simulink model "full_three_axis"  (R2026b)
settings: Solver=VariableStepAuto  StopTime=2
undefined symbols (not defined in the file): Bambient, k, T_threshold, Vmax
libraries: stm32f4xxblockslib x20, simulink x3, slpidlib x3, stm32blockslib x2, stm32g4xxblockslib x2
settings Model: STM32="{\"PWMOutput\":[{\"ID\":\"308\"},{\"ID\":\"321\"},{\"ID\":\"322\"}],\"UARTRead\":{\"ID\":\"291\"},\"AnalogInput\":{\"ID\":\"326\"},\"DigitalPortRead\":[{\"ID\":\"328\"},{\"ID\":\"404\"},{\"ID\":\"509\"},{\"ID\":\"514\"},{\"ID\":\"520\"},{\"ID\":\"525\"}],\"DigitalPortWrite\":[{\"ID\":\"353\"},{\"ID\":\"325\"},{\"ID\":\"370\"},{\"ID\":\"495\"},{\"ID\":\"497\"},{\"ID\":\"519\"},{\"ID\":\"530\"},{\"ID\":\"532\"},{\"ID\":\"534\"}],\"HardwareInterrupt\":[{\"ID\":\"333\"},{\"ID\":\"334\"}],\"UARTWrite\":{\"ID\":\"545\"}}"  Creator=Samuel  LastModifiedBy=Samuel
settings SimscapeCC: SimscapeUseEnergyAccounting=off

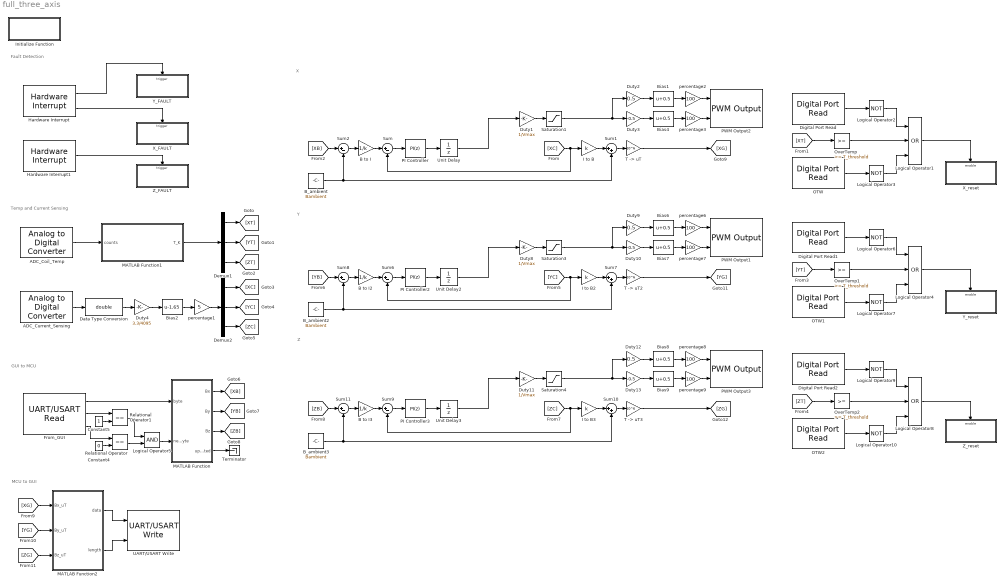
== system full_three_axis ==
  note: MCU to GUI
  note: Z
  note: Y
  note: X
  note: GUI to MCU
  note: Fault Detection
  note: Temp and Current Sensing
  ADC_Coil_Temp : stm32f4xxblockslib/Analog to Digital Converter  ADCModule=ADC2  ConversionGroup=Regular  TriggerMode=Trigger and read  NumberOfConversions=3  EnableBufferConv=off  BufferLength=1  OutputStatus=off  SampleTime=0.001  EnableSimPort=off  hoistedMaskSrc=ECSoC/ECSimCodegen/Analog to Digital Converter
  ADC_Current_Sensing : stm32f4xxblockslib/Analog to Digital Converter  ADCModule=ADC1  ConversionGroup=Regular  TriggerMode=Trigger and read  NumberOfConversions=3  EnableBufferConv=off  BufferLength=1  OutputStatus=off  SampleTime=0.001  EnableSimPort=off  hoistedMaskSrc=ECSoC/ECSimCodegen/Analog to Digital Converter
  B to I : Gain  Gain=1/k
  B to I2 : Gain  Gain=1/k
  B to I3 : Gain  Gain=1/k
  B_ambient : Constant  Value=Bambient
  B_ambient2 : Constant  Value=Bambient
  B_ambient3 : Constant  Value=Bambient
  Bias{1,4,6..9} (6 alike) : Bias  Bias=0.5  SaturateOnIntegerOverflow=off
  Bias2 : Bias  Bias=-1.65  SaturateOnIntegerOverflow=off
  Constant4 : Constant  Value=0
  Constant5 : Constant
  Data Type Conversion : DataTypeConversion  OutDataTypeStr=double  SaturateOnIntegerOverflow=off  RndMeth=Floor
  Demux1 : Demux  Outputs=3
  Demux2 : Demux  Outputs=3
  Digital Port Read : stm32f4xxblockslib/Digital Port Read  PortName=GPIOB  PinNumber=12  ReadOperation=on  IOAsArray=off  SampleTime=0.001  EnableSimPort=off  hoistedMaskSrc=ECSoC/ECSimCodegen/Digital Port Read
      settings: LibrarySourceBlock=stm32g4xxblockslib/Digital Port Read
  Digital Port Read1 : stm32f4xxblockslib/Digital Port Read  PortName=GPIOB  PinNumber=15  ReadOperation=on  IOAsArray=off  SampleTime=0.001  EnableSimPort=off  hoistedMaskSrc=ECSoC/ECSimCodegen/Digital Port Read
      settings: LibrarySourceBlock=stm32g4xxblockslib/Digital Port Read
  Digital Port Read2 : stm32f4xxblockslib/Digital Port Read  PortName=GPIOB  PinNumber=2  ReadOperation=on  IOAsArray=off  SampleTime=0.001  EnableSimPort=off  hoistedMaskSrc=ECSoC/ECSimCodegen/Digital Port Read
      settings: LibrarySourceBlock=stm32g4xxblockslib/Digital Port Read
  Duty1 : Gain  Gain=1/Vmax
  Duty10 : Gain  Gain=-0.5
  Duty11 : Gain  Gain=1/Vmax
  Duty12 : Gain  Gain=0.5
  Duty13 : Gain  Gain=-0.5
  Duty2 : Gain  Gain=0.5
  Duty3 : Gain  Gain=-0.5
  Duty4 : Gain  Gain=3.3/4095
  Duty8 : Gain  Gain=1/Vmax
  Duty9 : Gain  Gain=0.5
  From_GUI : stm32blockslib/UART//USART Read  UARTModule=LPUART1  DataType=uint8  DataLength=1  BlockingMode=off  BlockingTimeout=0.1  OutputLength=on  OutputStatus=on  SampleTime=0.001
  Hardware Interrupt : stm32g4xxblockslib/Hardware Interrupt  ISRGroup=External interrupts (EXTI)  ISRName=EXTI15_10_IRQHandler  ISRFunctionName=EXTI15_10_IRQHandler  ISRNumber=55  TaskPriority=30  EventsList={ 'on', 'EXTI15 Event', '1', 'inherit', 'off'; 'off', 'EXTI14 Event', '2', 'inherit', 'off'; 'off', 'EXTI13 Event', '3', 'inherit', 'off'; 'on', 'EXTI12 Event', '4', 'inherit', 'off'; 'off', 'EXTI11 Event', '5', 'inherit', 'off'; 'off', 'EXTI10 Event', '6', 'inherit', 'off'; 'off', 'Custom event', '7', 'inherit', 'off' }  SelectedEvents={'EXTI15 Event','EXTI12 Event'}  InternalTaskPriority=30  DisablePreemption=off  ClearInterruptFlagsAtEndOfEvent=on  InterruptDefinitionFile=$(TARGET_ROOT)/registry/interrupts/STM32F4xxBased_interrupts.xml  HardwareBoard=STM32G4xx Based  EnableSimPort=off
  Hardware Interrupt1 : stm32g4xxblockslib/Hardware Interrupt  ISRGroup=External interrupts (EXTI)  ISRName=EXTI2_IRQHandler  ISRFunctionName=EXTI2_IRQHandler  ISRNumber=23  TaskPriority=30  EventsList={ 'on', 'EXTI2 Event', '1', 'inherit', 'off'; 'off', 'Custom event', '2', 'inherit', 'off' }  SelectedEvents={'EXTI2 Event'}  InternalTaskPriority=30  DisablePreemption=off  ClearInterruptFlagsAtEndOfEvent=on  InterruptDefinitionFile=$(TARGET_ROOT)/registry/interrupts/STM32F4xxBased_interrupts.xml  HardwareBoard=STM32G4xx Based  EnableSimPort=off
  I to B : Gain  Gain=k
  I to B2 : Gain  Gain=k
  I to B3 : Gain  Gain=k
  Initialize Function : Subsystem  TreatAsAtomicUnit=on
  Logical Operator1 : Logic  Operator=OR  Inputs=3  AllPortsSameDT=off  OutDataTypeStr=boolean
  Logical Operator{2..3,6..7,9..10} (6 alike) : Logic  Operator=NOT  AllPortsSameDT=off  OutDataTypeStr=boolean
  Logical Operator4 : Logic  Operator=OR  Inputs=3  AllPortsSameDT=off  OutDataTypeStr=boolean
  Logical Operator5 : Logic  AllPortsSameDT=off  OutDataTypeStr=boolean
  Logical Operator8 : Logic  Operator=OR  Inputs=3  AllPortsSameDT=off  OutDataTypeStr=boolean
  MATLAB Function : MATLAB Function  TreatAsAtomicUnit=on
  MATLAB Function1 : MATLAB Function  TreatAsAtomicUnit=on
  MATLAB Function2 : MATLAB Function  TreatAsAtomicUnit=on
  OTW : stm32f4xxblockslib/Digital Port Read  PortName=GPIOB  PinNumber=11  ReadOperation=on  IOAsArray=off  SampleTime=0.001  EnableSimPort=off  hoistedMaskSrc=ECSoC/ECSimCodegen/Digital Port Read
      settings: LibrarySourceBlock=stm32g4xxblockslib/Digital Port Read
  OTW1 : stm32f4xxblockslib/Digital Port Read  PortName=GPIOB  PinNumber=14  ReadOperation=on  IOAsArray=off  SampleTime=0.001  EnableSimPort=off  hoistedMaskSrc=ECSoC/ECSimCodegen/Digital Port Read
      settings: LibrarySourceBlock=stm32g4xxblockslib/Digital Port Read
  OTW2 : stm32f4xxblockslib/Digital Port Read  PortName=GPIOB  PinNumber=1  ReadOperation=on  IOAsArray=off  SampleTime=0.001  EnableSimPort=off  hoistedMaskSrc=ECSoC/ECSimCodegen/Digital Port Read
      settings: LibrarySourceBlock=stm32g4xxblockslib/Digital Port Read
  OverTemp : simulink/Logic and Bit Operations/Compare To Constant  relop=>=  const=T_threshold  OutDataTypeStr=boolean
  OverTemp1 : simulink/Logic and Bit Operations/Compare To Constant  relop=>=  const=T_threshold  OutDataTypeStr=boolean
  OverTemp2 : simulink/Logic and Bit Operations/Compare To Constant  relop=>=  const=T_threshold  OutDataTypeStr=boolean
  PI Controller : slpidlib/PID Controller  Controller=PI  Form=Parallel  TimeDomain=Discrete-time  UseExternalTs=off  SampleTime=1e-4  IntegratorMethod=Forward Euler  FilterMethod=Forward Euler  ControllerParametersSource=internal  P=5  I=200  UseKiTs=off  D=0  UseExternalDerivativeSource=off  N=100  UseFilter=on  TunerSelectOption=Transfer Function Based (PID Tuner App)  InitialConditionSource=internal  InitialConditionForIntegrator=0  InitialConditionForFilter=0  DifferentiatorICPrevScaledInput=0  ExternalReset=none  TrackingMode=off  Kt=1  LimitOutput=on  SatLimitsSource=internal  UpperSaturationLimit=30  LowerSaturationLimit=-30  LinearizeAsGain=on  AntiWindupMode=clamping  Kb=1  LimitIntegrator=off  UpperIntegratorSaturationLimit=inf  LowerIntegratorSaturationLimit=-inf  POutMin=[]  POutMax=[]  IOutMin=[]  IOutMax=[]  DOutMin=[]  DOutMax=[]  NOutMin=[]  NOutMax=[]  SumOutMin=[]  SumOutMax=[]  SaturationOutMin=[]  SaturationOutMax=[]  PParamMin=[]  PParamMax=[]  IParamMin=[]  IParamMax=[]  DParamMin=[]  DParamMax=[]  NParamMin=[]  NParamMax=[]  KbParamMin=[]  KbParamMax=[]  KtParamMin=[]  KtParamMax=[]  KbOutMin=[]  KbOutMax=[]  KtOutMin=[]  KtOutMax=[]  IntegratorOutMin=[]  IntegratorOutMax=[]  FilterOutMin=[]  FilterOutMax=[]  SumI1OutMin=[]  SumI1OutMax=[]  SumI2OutMin=[]  SumI2OutMax=[]  SumI3OutMin=[]  SumI3OutMax=[]  SumI4OutMin=[]  SumI4OutMax=[]  SumDOutMin=[]  SumDOutMax=[]  DifferentiatorOutMin=[]  DifferentiatorOutMax=[]  FilterDiffOutCoefMin=[]  FilterDiffOutCoefMax=[]  ReciprocalOutMin=[]  ReciprocalOutMax=[]  SumDenOutMin=[]  SumDenOutMax=[]  SumNumOutMin=[]  SumNumOutMax=[]  DivideOutMin=[]  DivideOutMax=[]  UdiffTsProdOutMin=[]  UdiffTsProdOutMax=[]  NTsProdOutMin=[]  NTsProdOutMax=[]  UintegralTsProdOutMin=[]  UintegralTsProdOutMax=[]  UngainTsProdOutMin=[]  UngainTsProdOutMax=[]  ClampingZeroOutDataTypeStr=Inherit: Inherit via back propagation  ClampingZeroOutMin=[]  ClampingZeroOutMax=[]  FilterDenConstantOutDataTypeStr=Inherit: Inherit via back propagation  FilterDenConstantOutMin=[]  FilterDenConstantOutMax=[]  PCopyOutDataTypeStr=Inherit: Inherit via back propagation  PCopyOutMin=[]  PCopyOutMax=[]  NCopyOutDataTypeStr=Inherit: Inherit via back propagation  NCopyOutMin=[]  NCopyOutMax=[]  IntegratorContinuousStateAttributes=''  IntegratorStateMustResolveToSignalObject=off  IntegratorRTWStateStorageClass=Auto  FilterContinuousStateAttributes=''  FilterStateMustResolveToSignalObject=off  FilterRTWStateStorageClass=Auto  ParallelPVariant=InternalParameters  IdealPVariant=Disabled  IVariant=InternalParameters  DVariant=Disabled  IntegratorVariant=Discrete  SatVariant=Enabled  AWVariant=DiscClampingParallel  PCopyVariant=Disabled  TRVariant=Disabled  FdbkBlocksVariant=Forward  IdealPFdbkVariant=Disabled  SatFdbkVariant=Disabled  DerivativeFilterVariant=Disabled  NVariant=Disabled  NCopyVariant=Disabled_SignalSpec  FilterICVariant=Disabled  IntegratorICVariant=InternalICs  ExternalResetVariant=Disabled  TRSumVariant=Passthrough  SumFdbkVariant=Disabled  SumVariant=Sum_PI  TsampFilterVariant=InternalTs  TsampNgainVariant=Passthrough  TsampIntegralVariant=Disabled_SignalSpec  ExternalSaturationOutDataTypeStr=Inherit: Same as second input  DerivativeSourceVariant=Disabled  PreIntVariant=InternalPreInt
  PI Controller2 : slpidlib/PID Controller  Controller=PI  Form=Parallel  TimeDomain=Discrete-time  UseExternalTs=off  SampleTime=1e-4  IntegratorMethod=Forward Euler  FilterMethod=Forward Euler  ControllerParametersSource=internal  P=5  I=200  UseKiTs=off  D=0  UseExternalDerivativeSource=off  N=100  UseFilter=on  TunerSelectOption=Transfer Function Based (PID Tuner App)  InitialConditionSource=internal  InitialConditionForIntegrator=0  InitialConditionForFilter=0  DifferentiatorICPrevScaledInput=0  ExternalReset=none  TrackingMode=off  Kt=1  LimitOutput=on  SatLimitsSource=internal  UpperSaturationLimit=30  LowerSaturationLimit=-30  LinearizeAsGain=on  AntiWindupMode=clamping  Kb=1  LimitIntegrator=off  UpperIntegratorSaturationLimit=inf  LowerIntegratorSaturationLimit=-inf  POutMin=[]  POutMax=[]  IOutMin=[]  IOutMax=[]  DOutMin=[]  DOutMax=[]  NOutMin=[]  NOutMax=[]  SumOutMin=[]  SumOutMax=[]  SaturationOutMin=[]  SaturationOutMax=[]  PParamMin=[]  PParamMax=[]  IParamMin=[]  IParamMax=[]  DParamMin=[]  DParamMax=[]  NParamMin=[]  NParamMax=[]  KbParamMin=[]  KbParamMax=[]  KtParamMin=[]  KtParamMax=[]  KbOutMin=[]  KbOutMax=[]  KtOutMin=[]  KtOutMax=[]  IntegratorOutMin=[]  IntegratorOutMax=[]  FilterOutMin=[]  FilterOutMax=[]  SumI1OutMin=[]  SumI1OutMax=[]  SumI2OutMin=[]  SumI2OutMax=[]  SumI3OutMin=[]  SumI3OutMax=[]  SumI4OutMin=[]  SumI4OutMax=[]  SumDOutMin=[]  SumDOutMax=[]  DifferentiatorOutMin=[]  DifferentiatorOutMax=[]  FilterDiffOutCoefMin=[]  FilterDiffOutCoefMax=[]  ReciprocalOutMin=[]  ReciprocalOutMax=[]  SumDenOutMin=[]  SumDenOutMax=[]  SumNumOutMin=[]  SumNumOutMax=[]  DivideOutMin=[]  DivideOutMax=[]  UdiffTsProdOutMin=[]  UdiffTsProdOutMax=[]  NTsProdOutMin=[]  NTsProdOutMax=[]  UintegralTsProdOutMin=[]  UintegralTsProdOutMax=[]  UngainTsProdOutMin=[]  UngainTsProdOutMax=[]  ClampingZeroOutDataTypeStr=Inherit: Inherit via back propagation  ClampingZeroOutMin=[]  ClampingZeroOutMax=[]  FilterDenConstantOutDataTypeStr=Inherit: Inherit via back propagation  FilterDenConstantOutMin=[]  FilterDenConstantOutMax=[]  PCopyOutDataTypeStr=Inherit: Inherit via back propagation  PCopyOutMin=[]  PCopyOutMax=[]  NCopyOutDataTypeStr=Inherit: Inherit via back propagation  NCopyOutMin=[]  NCopyOutMax=[]  IntegratorContinuousStateAttributes=''  IntegratorStateMustResolveToSignalObject=off  IntegratorRTWStateStorageClass=Auto  FilterContinuousStateAttributes=''  FilterStateMustResolveToSignalObject=off  FilterRTWStateStorageClass=Auto  ParallelPVariant=InternalParameters  IdealPVariant=Disabled  IVariant=InternalParameters  DVariant=Disabled  IntegratorVariant=Discrete  SatVariant=Enabled  AWVariant=DiscClampingParallel  PCopyVariant=Disabled  TRVariant=Disabled  FdbkBlocksVariant=Forward  IdealPFdbkVariant=Disabled  SatFdbkVariant=Disabled  DerivativeFilterVariant=Disabled  NVariant=Disabled  NCopyVariant=Disabled_SignalSpec  FilterICVariant=Disabled  IntegratorICVariant=InternalICs  ExternalResetVariant=Disabled  TRSumVariant=Passthrough  SumFdbkVariant=Disabled  SumVariant=Sum_PI  TsampFilterVariant=InternalTs  TsampNgainVariant=Passthrough  TsampIntegralVariant=Disabled_SignalSpec  ExternalSaturationOutDataTypeStr=Inherit: Same as second input  DerivativeSourceVariant=Disabled  PreIntVariant=InternalPreInt
  PI Controller3 : slpidlib/PID Controller  Controller=PI  Form=Parallel  TimeDomain=Discrete-time  UseExternalTs=off  SampleTime=1e-4  IntegratorMethod=Forward Euler  FilterMethod=Forward Euler  ControllerParametersSource=internal  P=5  I=200  UseKiTs=off  D=0  UseExternalDerivativeSource=off  N=100  UseFilter=on  TunerSelectOption=Transfer Function Based (PID Tuner App)  InitialConditionSource=internal  InitialConditionForIntegrator=0  InitialConditionForFilter=0  DifferentiatorICPrevScaledInput=0  ExternalReset=none  TrackingMode=off  Kt=1  LimitOutput=on  SatLimitsSource=internal  UpperSaturationLimit=30  LowerSaturationLimit=-30  LinearizeAsGain=on  AntiWindupMode=clamping  Kb=1  LimitIntegrator=off  UpperIntegratorSaturationLimit=inf  LowerIntegratorSaturationLimit=-inf  POutMin=[]  POutMax=[]  IOutMin=[]  IOutMax=[]  DOutMin=[]  DOutMax=[]  NOutMin=[]  NOutMax=[]  SumOutMin=[]  SumOutMax=[]  SaturationOutMin=[]  SaturationOutMax=[]  PParamMin=[]  PParamMax=[]  IParamMin=[]  IParamMax=[]  DParamMin=[]  DParamMax=[]  NParamMin=[]  NParamMax=[]  KbParamMin=[]  KbParamMax=[]  KtParamMin=[]  KtParamMax=[]  KbOutMin=[]  KbOutMax=[]  KtOutMin=[]  KtOutMax=[]  IntegratorOutMin=[]  IntegratorOutMax=[]  FilterOutMin=[]  FilterOutMax=[]  SumI1OutMin=[]  SumI1OutMax=[]  SumI2OutMin=[]  SumI2OutMax=[]  SumI3OutMin=[]  SumI3OutMax=[]  SumI4OutMin=[]  SumI4OutMax=[]  SumDOutMin=[]  SumDOutMax=[]  DifferentiatorOutMin=[]  DifferentiatorOutMax=[]  FilterDiffOutCoefMin=[]  FilterDiffOutCoefMax=[]  ReciprocalOutMin=[]  ReciprocalOutMax=[]  SumDenOutMin=[]  SumDenOutMax=[]  SumNumOutMin=[]  SumNumOutMax=[]  DivideOutMin=[]  DivideOutMax=[]  UdiffTsProdOutMin=[]  UdiffTsProdOutMax=[]  NTsProdOutMin=[]  NTsProdOutMax=[]  UintegralTsProdOutMin=[]  UintegralTsProdOutMax=[]  UngainTsProdOutMin=[]  UngainTsProdOutMax=[]  ClampingZeroOutDataTypeStr=Inherit: Inherit via back propagation  ClampingZeroOutMin=[]  ClampingZeroOutMax=[]  FilterDenConstantOutDataTypeStr=Inherit: Inherit via back propagation  FilterDenConstantOutMin=[]  FilterDenConstantOutMax=[]  PCopyOutDataTypeStr=Inherit: Inherit via back propagation  PCopyOutMin=[]  PCopyOutMax=[]  NCopyOutDataTypeStr=Inherit: Inherit via back propagation  NCopyOutMin=[]  NCopyOutMax=[]  IntegratorContinuousStateAttributes=''  IntegratorStateMustResolveToSignalObject=off  IntegratorRTWStateStorageClass=Auto  FilterContinuousStateAttributes=''  FilterStateMustResolveToSignalObject=off  FilterRTWStateStorageClass=Auto  ParallelPVariant=InternalParameters  IdealPVariant=Disabled  IVariant=InternalParameters  DVariant=Disabled  IntegratorVariant=Discrete  SatVariant=Enabled  AWVariant=DiscClampingParallel  PCopyVariant=Disabled  TRVariant=Disabled  FdbkBlocksVariant=Forward  IdealPFdbkVariant=Disabled  SatFdbkVariant=Disabled  DerivativeFilterVariant=Disabled  NVariant=Disabled  NCopyVariant=Disabled_SignalSpec  FilterICVariant=Disabled  IntegratorICVariant=InternalICs  ExternalResetVariant=Disabled  TRSumVariant=Passthrough  SumFdbkVariant=Disabled  SumVariant=Sum_PI  TsampFilterVariant=InternalTs  TsampNgainVariant=Passthrough  TsampIntegralVariant=Disabled_SignalSpec  ExternalSaturationOutDataTypeStr=Inherit: Same as second input  DerivativeSourceVariant=Disabled  PreIntVariant=InternalPreInt
  PWM Output1 : stm32f4xxblockslib/PWM Output  ProcessorFamily=STM32G4  TimerModule=TIM1  DutycycleUnits=Percentage  EnableChannel1=off  EnableCaptureCompare1Input=off  EnableCaptureCompare1ComplementaryInput=off  EnableOutputCompare1ModeInput=off  EnableChannel2=off  EnableCaptureCompare2Input=off  EnableCaptureCompare2ComplementaryInput=off  EnableOutputCompare2ModeInput=off  EnableChannel3=on  EnableCaptureCompare3Input=off  EnableCaptureCompare3ComplementaryInput=off  EnableOutputCompare3ModeInput=off  EnableChannel4=on  EnableCaptureCompare4Input=off  EnableCaptureCompare4ComplementaryInput=off  EnableOutputCompare4ModeInput=off  EnableChannel5=off  EnableCaptureCompare5Input=off  EnableOutputCompare5ModeInput=off  EnableChannel6=off  EnableCaptureCompare6Input=off  EnableOutputCompare6ModeInput=off  EnableCounterInput=off  EnableMainOutputInput=off  EnableFrequencyInput=off  SetRCAfterCE=off  OutputDirection=off  OutputMainOutputEnableStatus=off  SampleTime=0.1  EnableSimPort=off  EnableUpdateEvent=off  EnableCaptureCompare1Event=off  EnableCaptureCompare2Event=off  EnableCaptureCompare3Event=off  EnableCaptureCompare4Event=off  EnableTriggerEvent=off  EnableBreakEvent=off  EnableBreakEvent2=off  hoistedMaskSrc=ECSoC/ECSimCodegen/PWM Output
      settings: LibrarySourceBlock=stm32g4xxblockslib/PWM Output
  PWM Output2 : stm32f4xxblockslib/PWM Output  ProcessorFamily=STM32G4  TimerModule=TIM1  DutycycleUnits=Percentage  EnableChannel1=on  EnableCaptureCompare1Input=off  EnableCaptureCompare1ComplementaryInput=off  EnableOutputCompare1ModeInput=off  EnableChannel2=on  EnableCaptureCompare2Input=off  EnableCaptureCompare2ComplementaryInput=off  EnableOutputCompare2ModeInput=off  EnableChannel3=off  EnableCaptureCompare3Input=off  EnableCaptureCompare3ComplementaryInput=off  EnableOutputCompare3ModeInput=off  EnableChannel4=off  EnableCaptureCompare4Input=off  EnableCaptureCompare4ComplementaryInput=off  EnableOutputCompare4ModeInput=off  EnableChannel5=off  EnableCaptureCompare5Input=off  EnableOutputCompare5ModeInput=off  EnableChannel6=off  EnableCaptureCompare6Input=off  EnableOutputCompare6ModeInput=off  EnableCounterInput=off  EnableMainOutputInput=off  EnableFrequencyInput=off  SetRCAfterCE=off  OutputDirection=off  OutputMainOutputEnableStatus=off  SampleTime=0.1  EnableSimPort=off  EnableUpdateEvent=off  EnableCaptureCompare1Event=off  EnableCaptureCompare2Event=off  EnableCaptureCompare3Event=off  EnableCaptureCompare4Event=off  EnableTriggerEvent=off  EnableBreakEvent=off  EnableBreakEvent2=off  hoistedMaskSrc=ECSoC/ECSimCodegen/PWM Output
      settings: LibrarySourceBlock=stm32g4xxblockslib/PWM Output
  PWM Output3 : stm32f4xxblockslib/PWM Output  ProcessorFamily=STM32G4  TimerModule=TIM8  DutycycleUnits=Percentage  EnableChannel1=on  EnableCaptureCompare1Input=off  EnableCaptureCompare1ComplementaryInput=off  EnableOutputCompare1ModeInput=off  EnableChannel2=on  EnableCaptureCompare2Input=off  EnableCaptureCompare2ComplementaryInput=off  EnableOutputCompare2ModeInput=off  EnableChannel3=off  EnableCaptureCompare3Input=off  EnableCaptureCompare3ComplementaryInput=off  EnableOutputCompare3ModeInput=off  EnableChannel4=off  EnableCaptureCompare4Input=off  EnableCaptureCompare4ComplementaryInput=off  EnableOutputCompare4ModeInput=off  EnableChannel5=off  EnableCaptureCompare5Input=off  EnableOutputCompare5ModeInput=off  EnableChannel6=off  EnableCaptureCompare6Input=off  EnableOutputCompare6ModeInput=off  EnableCounterInput=off  EnableMainOutputInput=off  EnableFrequencyInput=off  SetRCAfterCE=off  OutputDirection=off  OutputMainOutputEnableStatus=off  SampleTime=0.1  EnableSimPort=off  EnableUpdateEvent=off  EnableCaptureCompare1Event=off  EnableCaptureCompare2Event=off  EnableCaptureCompare3Event=off  EnableCaptureCompare4Event=off  EnableTriggerEvent=off  EnableBreakEvent=off  EnableBreakEvent2=off  hoistedMaskSrc=ECSoC/ECSimCodegen/PWM Output
      settings: LibrarySourceBlock=stm32g4xxblockslib/PWM Output
  Relational Operator : RelationalOperator  Operator===  OutDataTypeStr=boolean  RndMeth=Simplest  InputSameDT=off
  Relational Operator1 : RelationalOperator  Operator===  OutDataTypeStr=boolean  RndMeth=Simplest  InputSameDT=off
  Saturation1 : Saturate  UpperLimit=1  LowerLimit=-1
  Saturation3 : Saturate  UpperLimit=1  LowerLimit=-1
  Saturation4 : Saturate  UpperLimit=1  LowerLimit=-1
  Sum{,2,6,8..9,11} (6 alike) : Sum  Inputs=|+-
  Sum1 : Sum  Inputs=|++
  Sum10 : Sum  Inputs=|++
  Sum7 : Sum  Inputs=|++
  "T -> uT" : Gain  Gain=10^6
  "T -> uT2" : Gain  Gain=10^6
  "T -> uT3" : Gain  Gain=10^6
  Terminator : Terminator
  UART/USART Write : stm32blockslib/UART//USART Write  UARTModule=LPUART1  LengthOfDataToSend=on  BlockingMode=off  BlockingTimeout=0.1  OutputStatus=off
  Unit Delay : UnitDelay  SampleTime=1e-4
  Unit Delay2 : UnitDelay  SampleTime=1e-4
  Unit Delay3 : UnitDelay  SampleTime=1e-4
  X_FAULT : Subsystem  TreatAsAtomicUnit=on
  X_reset : Subsystem  TreatAsAtomicUnit=on
  Y_FAULT : Subsystem  TreatAsAtomicUnit=on
  Y_reset : Subsystem  TreatAsAtomicUnit=on
  Z_FAULT : Subsystem  TreatAsAtomicUnit=on
  Z_reset : Subsystem  TreatAsAtomicUnit=on
  percentage1 : Gain  Gain=5
  percentage{2..3,6..9} (6 alike) : Gain  Gain=100
  wires:
  Sum/1 -> PI Controller/1
  B_ambient/1 -> Sum1/2, Sum2/2
  Sum2/1 -> B to I/1
  B to I/1 -> Sum/1
  I to B/1 -> Sum1/1
  PI Controller/1 -> Unit Delay/1
  Sum1/1 -> "T -> uT"/1
  From_GUI/1 -> MATLAB Function/1(byte)
  Constant5/1 -> Relational Operator1/2
  Logical Operator5/1 -> MATLAB Function/2(newByte)
  Relational Operator1/1 -> Logical Operator5/1
  Relational Operator/1 -> Logical Operator5/2
  Constant4/1 -> Relational Operator/2
  From_GUI/2 -> Relational Operator1/1
  From_GUI/3 -> Relational Operator/1
  Unit Delay/1 -> Duty1/1
  Duty1/1 -> Saturation1/1
  Saturation1/1 -> Duty2/1, Duty3/1
  Bias4/1 -> percentage3/1
  Bias1/1 -> percentage2/1
  Duty3/1 -> Bias4/1
  percentage2/1 -> PWM Output2/1
  percentage3/1 -> PWM Output2/2
  Duty2/1 -> Bias1/1
  ADC_Current_Sensing/1 -> Data Type Conversion/1
  "T -> uT"/1 -> [XG]
  Logical Operator1/1 -> X_reset/Enable
  OTW/1 -> Logical Operator3/1
  [XC] -> Sum/2, I to B/1
  Hardware Interrupt1/1 -> Z_FAULT/Trigger
  [XT] -> OverTemp/1
  MATLAB Function/1(Bx) -> [XB]
  MATLAB Function/2(By) -> [YB]
  MATLAB Function/3(Bz) -> [ZB]
  [XB] -> Sum2/1
  Hardware Interrupt/2 -> X_FAULT/Trigger
  Hardware Interrupt/1 -> Y_FAULT/Trigger
  Data Type Conversion/1 -> Duty4/1
  Duty4/1 -> Bias2/1
  Bias2/1 -> percentage1/1
  percentage1/1 -> Demux2/1
  Demux2/1 -> [XC]
  Demux2/2 -> [YC]
  Demux2/3 -> [ZC]
  Demux1/3 -> [ZT]
  Demux1/2 -> [YT]
  Demux1/1 -> [XT]
  ADC_Coil_Temp/1 -> MATLAB Function1/1(counts)
  MATLAB Function1/1(T_K) -> Demux1/1
  Logical Operator3/1 -> Logical Operator1/3
  OverTemp/1 -> Logical Operator1/2
  Digital Port Read/1 -> Logical Operator2/1
  Logical Operator2/1 -> Logical Operator1/1
  [YB] -> Sum8/1
  Duty8/1 -> Saturation3/1
  Saturation3/1 -> Duty9/1, Duty10/1
  Sum6/1 -> PI Controller2/1
  "T -> uT2"/1 -> [YG]
  B_ambient2/1 -> Sum7/2, Sum8/2
  PI Controller2/1 -> Unit Delay2/1
  I to B2/1 -> Sum7/1
  Sum8/1 -> B to I2/1
  percentage7/1 -> PWM Output1/2
  [YC] -> Sum6/2, I to B2/1
  Unit Delay2/1 -> Duty8/1
  Sum7/1 -> "T -> uT2"/1
  Duty9/1 -> Bias6/1
  Bias7/1 -> percentage7/1
  Duty10/1 -> Bias7/1
  B to I2/1 -> Sum6/1
  percentage6/1 -> PWM Output1/1
  Bias6/1 -> percentage6/1
  [ZB] -> Sum11/1
  Duty11/1 -> Saturation4/1
  Saturation4/1 -> Duty12/1, Duty13/1
  Sum9/1 -> PI Controller3/1
  "T -> uT3"/1 -> [ZG]
  B_ambient3/1 -> Sum10/2, Sum11/2
  PI Controller3/1 -> Unit Delay3/1
  I to B3/1 -> Sum10/1
  Sum11/1 -> B to I3/1
  percentage9/1 -> PWM Output3/2
  [ZC] -> Sum9/2, I to B3/1
  Unit Delay3/1 -> Duty11/1
  Sum10/1 -> "T -> uT3"/1
  Duty12/1 -> Bias8/1
  Bias9/1 -> percentage9/1
  Duty13/1 -> Bias9/1
  B to I3/1 -> Sum9/1
  percentage8/1 -> PWM Output3/1
  Bias8/1 -> percentage8/1
  Logical Operator7/1 -> Logical Operator4/3
  OverTemp1/1 -> Logical Operator4/2
  Digital Port Read1/1 -> Logical Operator6/1
  Logical Operator4/1 -> Y_reset/Enable
  [YT] -> OverTemp1/1
  OTW1/1 -> Logical Operator7/1
  Logical Operator6/1 -> Logical Operator4/1
  Digital Port Read2/1 -> Logical Operator9/1
  Logical Operator9/1 -> Logical Operator8/1
  [ZT] -> OverTemp2/1
  OverTemp2/1 -> Logical Operator8/2
  OTW2/1 -> Logical Operator10/1
  Logical Operator10/1 -> Logical Operator8/3
  Logical Operator8/1 -> Z_reset/Enable
  MATLAB Function/4(updated) -> Terminator/1
  [XG] -> MATLAB Function2/1(Bx_uT)
  [YG] -> MATLAB Function2/2(By_uT)
  [ZG] -> MATLAB Function2/3(Bz_uT)
  MATLAB Function2/1(data) -> UART/USART Write/1
  MATLAB Function2/2(length) -> UART/USART Write/2

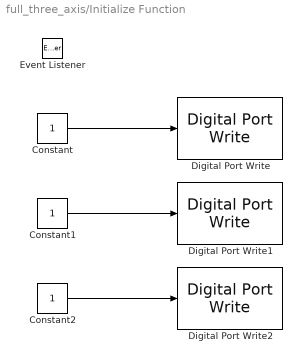
== system full_three_axis/Initialize Function ==
  Constant : Constant
  Constant1 : Constant
  Constant2 : Constant
  Digital Port Write : stm32f4xxblockslib/Digital Port Write  PortName=GPIOC  PinNumber=10  ReadOperation=off  IOAsArray=off  EnableSimPort=off  hoistedMaskSrc=ECSoC/ECSimCodegen/Digital Port Write
      settings: LibrarySourceBlock=stm32g4xxblockslib/Digital Port Write
  Digital Port Write1 : stm32f4xxblockslib/Digital Port Write  PortName=GPIOC  PinNumber=11  ReadOperation=off  IOAsArray=off  EnableSimPort=off  hoistedMaskSrc=ECSoC/ECSimCodegen/Digital Port Write
      settings: LibrarySourceBlock=stm32g4xxblockslib/Digital Port Write
  Digital Port Write2 : stm32f4xxblockslib/Digital Port Write  PortName=GPIOC  PinNumber=12  ReadOperation=off  IOAsArray=off  EnableSimPort=off  hoistedMaskSrc=ECSoC/ECSimCodegen/Digital Port Write
      settings: LibrarySourceBlock=stm32g4xxblockslib/Digital Port Write
  Event Listener : EventListener  DisableCoverage=on  EventName=reset
  wires:
  Constant/1 -> Digital Port Write/1
  Constant1/1 -> Digital Port Write1/1
  Constant2/1 -> Digital Port Write2/1

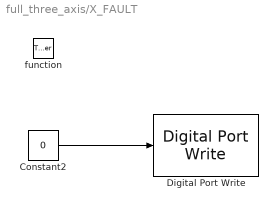
== system full_three_axis/X_FAULT ==
  function : TriggerPort  TriggerType=function-call  VariantControl=(inherit)
  Constant2 : Constant  Value=0
  Digital Port Write : stm32f4xxblockslib/Digital Port Write  PortName=GPIOC  PinNumber=10  ReadOperation=off  IOAsArray=off  EnableSimPort=off  hoistedMaskSrc=ECSoC/ECSimCodegen/Digital Port Write
      settings: LibrarySourceBlock=stm32g4xxblockslib/Digital Port Write
  wires:
  Constant2/1 -> Digital Port Write/1

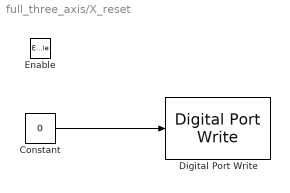
== system full_three_axis/X_reset ==
  Enable : EnablePort
  Constant : Constant  Value=0
  Digital Port Write : stm32f4xxblockslib/Digital Port Write  PortName=GPIOC  PinNumber=10  ReadOperation=off  IOAsArray=off  EnableSimPort=off  hoistedMaskSrc=ECSoC/ECSimCodegen/Digital Port Write
      settings: LibrarySourceBlock=stm32g4xxblockslib/Digital Port Write
  wires:
  Constant/1 -> Digital Port Write/1

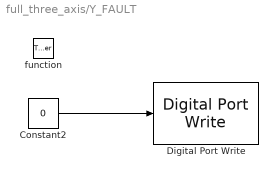
== system full_three_axis/Y_FAULT ==
  function : TriggerPort  TriggerType=function-call  VariantControl=(inherit)
  Constant2 : Constant  Value=0
  Digital Port Write : stm32f4xxblockslib/Digital Port Write  PortName=GPIOC  PinNumber=11  ReadOperation=off  IOAsArray=off  EnableSimPort=off  hoistedMaskSrc=ECSoC/ECSimCodegen/Digital Port Write
      settings: LibrarySourceBlock=stm32g4xxblockslib/Digital Port Write
  wires:
  Constant2/1 -> Digital Port Write/1

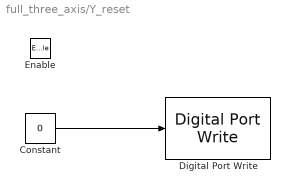
== system full_three_axis/Y_reset ==
  Enable : EnablePort
  Constant : Constant  Value=0
  Digital Port Write : stm32f4xxblockslib/Digital Port Write  PortName=GPIOC  PinNumber=11  ReadOperation=off  IOAsArray=off  EnableSimPort=off  hoistedMaskSrc=ECSoC/ECSimCodegen/Digital Port Write
      settings: LibrarySourceBlock=stm32g4xxblockslib/Digital Port Write
  wires:
  Constant/1 -> Digital Port Write/1

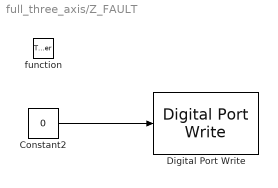
== system full_three_axis/Z_FAULT ==
  function : TriggerPort  TriggerType=function-call  VariantControl=(inherit)
  Constant2 : Constant  Value=0
  Digital Port Write : stm32f4xxblockslib/Digital Port Write  PortName=GPIOC  PinNumber=12  ReadOperation=off  IOAsArray=off  EnableSimPort=off  hoistedMaskSrc=ECSoC/ECSimCodegen/Digital Port Write
      settings: LibrarySourceBlock=stm32g4xxblockslib/Digital Port Write
  wires:
  Constant2/1 -> Digital Port Write/1

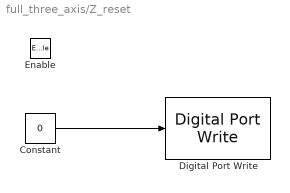
== system full_three_axis/Z_reset ==
  Enable : EnablePort
  Constant : Constant  Value=0
  Digital Port Write : stm32f4xxblockslib/Digital Port Write  PortName=GPIOC  PinNumber=12  ReadOperation=off  IOAsArray=off  EnableSimPort=off  hoistedMaskSrc=ECSoC/ECSimCodegen/Digital Port Write
      settings: LibrarySourceBlock=stm32g4xxblockslib/Digital Port Write
  wires:
  Constant/1 -> Digital Port Write/1

== matlab function full_three_axis/MATLAB Function1 ==
  data: counts input; T_K output
function T_K = ThermistorTemperature(counts)
%#codegen
R_fixed = 10000;  % Fixed resistor, ohms
R0      = 10000;  % NTC resistance at 25°C, ohms
T0      = 298.15; % Reference temperature, kelvin
Beta    = 3950;   % Replace with thermistor's actual Beta
ADC_max = 4095;

T_K = zeros(size(counts));

for i = 1:numel(counts)
    n = double(counts(i));

    % Avoid division by zero and log(0).
    n = min(max(n, 1), ADC_max - 1);

    R_ntc = R_fixed * n / (ADC_max - n);
    T_K(i) = 1 / (1/T0 + log(R_ntc/R0)/Beta);
end
end

== matlab function full_three_axis/MATLAB Function ==
  data: byte input; Bx output; newByte input; By output; Bz output; updated output
function [Bx, By, Bz, updated] = Decode_SET(byte, newByte)
%#codegen
% GUI field values are assumed to be in microtesla.

persistent buffer count dropping lastB

if isempty(count)
    buffer = repmat(' ', 1, 96);
    count = 0;
    dropping = false;
    lastB = zeros(3, 1);
end

updated = false;

if newByte
    if byte == uint8(10)              % Newline: end of command
        if ~dropping && count > 0
            [values, n] = sscanf( ...
                buffer, 'SET: %f , %f , %f', [3 1]);

            if n == 3
                if all(isfinite(values))
                    lastB = values * 1e-6; % microtesla -> tesla
                    updated = true;
                end
            end
        end

        buffer(:) = ' ';
        count = 0;
        dropping = false;

    elseif byte ~= uint8(13)          % Ignore carriage return
        if ~dropping
            if count < 96
                count = count + 1;
                buffer(count) = char(byte);
            else
                dropping = true;     % Discard oversized line
            end
        end
    end
end

Bx = lastB(1);
By = lastB(2);
Bz = lastB(3);
end

== matlab function full_three_axis/MATLAB Function2 ==
  data: Bx_uT input; data output; By_uT input; Bz_uT input; length output
function [data, length] = Format_GUI_Data(Bx_uT, By_uT, Bz_uT)
%#codegen

% Fixed-size UART output buffer.
data = zeros(1, 64, 'uint8');

% Scientific notation keeps message length bounded.
coder.varsize('message', [1 64], [0 1]);
message = sprintf('DATA:%.6e,%.6e,%.6e\n', ...
    double(Bx_uT), double(By_uT), double(Bz_uT));

length = uint8(numel(message));

for i = 1:numel(message)
    data(i) = uint8(message(i));
end
end
